simulink model "deep_fryer_adaptive_pid"  (R2024a)
settings: Solver=ode1  StartTime=0.0  StopTime=stop_time  FixedStep=dt  RelTol=1e-3
InitFcn:
  | if ~exist('tau','var'); tau = 180; end
  | if ~exist('L','var'); L = 10; end
  | if ~exist('K','var'); K = 1.9; end
  | if ~exist('T_ambient','var'); T_ambient = 30; end
  | if ~exist('Kp0','var'); Kp0 = 2; end
  | if ~exist('Ki0','var'); Ki0 = 0.05; end
  | if ~exist('Kd0','var'); Kd0 = 0.5; end
  | if ~exist('lambda_p','var'); lambda_p = 0.02; end
  | if ~exist('lambda_i','var'); lambda_i = 0.001; end
  | if ~exist('lambda_d','var'); lambda_d = 0.01; end
  | if ~exist('Kp_max','var'); Kp_max = 10; end
  | if ~exist('Ki_max','var'); Ki_max = 1; end
  | if ~exist('Kd_max','var'); Kd_max = 5; end
  | if ~exist('Tf_deriv','var'); Tf_deriv = 5; end
  | if ~exist('dead_hi','var'); dead_hi = 1.5; end
  | if ~exist('dead_lo','var'); dead_lo = 0.75; end
  | if ~exist('taper','var'); taper = 1; end
  | if ~exist('n_avg','var'); n_avg = 1; end
  | if ~exist('out_min','var'); out_min = 0; end
  | if ~exist('out_max','var'); out_max = 100; end
  | if ~exist('servo_tau','var'); servo_tau = 0.7; end
  | if ~exist('dt','var'); dt = 1; end
  | if ~exist('stop_time','var'); stop_time = 1800; end
  | if ~exist('Tref_value','var'); Tref_value = 150; end
values from neighbouring files (symbols this model uses):
  dead_hi = 1.5    [build_deep_fryer_model.m]
  dead_lo = 0.75    [build_deep_fryer_model.m]
  dt = 1    [build_deep_fryer_model.m]
  K = 1.9    [build_deep_fryer_model.m]
  Kd0 = 0.5    [build_deep_fryer_model.m]
  Kd_max = 5    [build_deep_fryer_model.m]
  Ki0 = 0.05    [build_deep_fryer_model.m]
  Ki_max = 1    [build_deep_fryer_model.m]
  Kp0 = 2    [build_deep_fryer_model.m]
  Kp_max = 10    [build_deep_fryer_model.m]
  L = 10    [build_deep_fryer_model.m]
  lambda_d = 0.01    [build_deep_fryer_model.m]
  lambda_i = 0.001    [build_deep_fryer_model.m]
  lambda_p = 0.02    [build_deep_fryer_model.m]
  n_avg = 1    [build_deep_fryer_model.m]
  out_max = 100    [build_deep_fryer_model.m]
  out_min = 0    [build_deep_fryer_model.m]
  servo_tau = 0.7    [build_deep_fryer_model.m]
  T_ambient = 30    [build_deep_fryer_model.m]
  taper = 1.0    (= 1)    [build_deep_fryer_model.m]
  tau = 180    [build_deep_fryer_model.m]
  Tf_deriv = 5    [build_deep_fryer_model.m]
  Tref_value = 150    [build_deep_fryer_model.m]
settings Model: Creator=indie  LastModifiedBy=indie

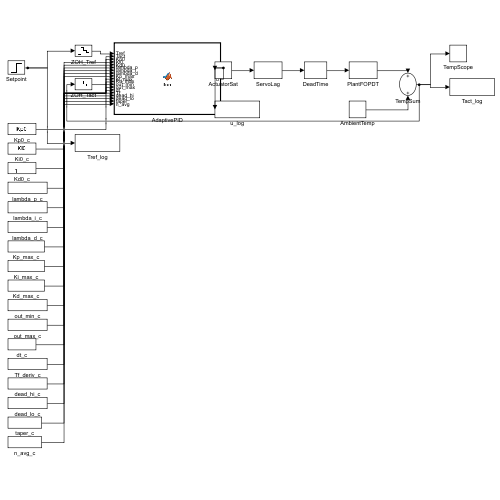
[thumbnail: Simulink's stored preview of the top-level diagram]
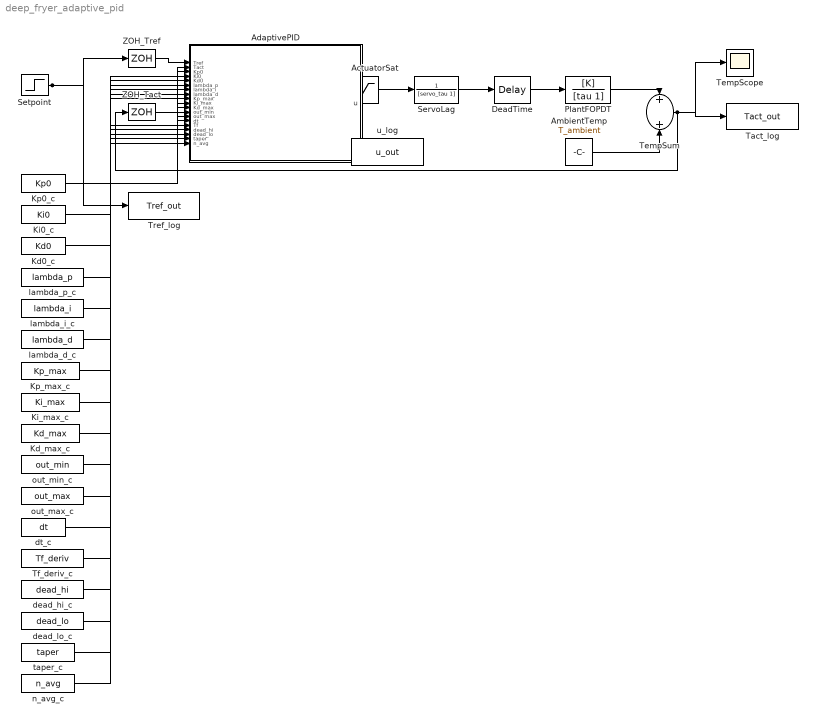
== system deep_fryer_adaptive_pid ==
  ActuatorSat : Saturate  UpperLimit=out_max  LowerLimit=out_min
  AdaptivePID : MATLAB Function  TreatAsAtomicUnit=on
  AmbientTemp : Constant  Value=T_ambient
  DeadTime : TransportDelay  DelayTime=L
  Kd0_c : Constant  Value=Kd0
  Kd_max_c : Constant  Value=Kd_max
  Ki0_c : Constant  Value=Ki0
  Ki_max_c : Constant  Value=Ki_max
  Kp0_c : Constant  Value=Kp0
  Kp_max_c : Constant  Value=Kp_max
  PlantFOPDT : TransferFcn  Numerator=[K]  Denominator=[tau 1]
  ServoLag : TransferFcn  Denominator=[servo_tau 1]
  Setpoint : Step  Time=0  Before=Tref_value  After=Tref_value  SampleTime=0
  Tact_log : ToWorkspace  VariableName=Tact_out  SaveFormat=Structure With Time  SampleTime=-1
  TempScope : Scope
  TempSum : Sum
  Tf_deriv_c : Constant  Value=Tf_deriv
  Tref_log : ToWorkspace  VariableName=Tref_out  SaveFormat=Structure With Time  SampleTime=-1
  ZOH_Tact : ZeroOrderHold  SampleTime=dt
  ZOH_Tref : ZeroOrderHold  SampleTime=dt
  dead_hi_c : Constant  Value=dead_hi
  dead_lo_c : Constant  Value=dead_lo
  dt_c : Constant  Value=dt
  lambda_d_c : Constant  Value=lambda_d
  lambda_i_c : Constant  Value=lambda_i
  lambda_p_c : Constant  Value=lambda_p
  n_avg_c : Constant  Value=n_avg
  out_max_c : Constant  Value=out_max
  out_min_c : Constant  Value=out_min
  taper_c : Constant  Value=taper
  u_log : ToWorkspace  VariableName=u_out  SaveFormat=Structure With Time  SampleTime=-1
  wires:
  ActuatorSat/1 -> ServoLag/1
  ServoLag/1 -> DeadTime/1
  DeadTime/1 -> PlantFOPDT/1
  PlantFOPDT/1 -> TempSum/1
  AmbientTemp/1 -> TempSum/2
  TempSum/1 -> TempScope/1, Tact_log/1, ZOH_Tact/1
  Setpoint/1 -> Tref_log/1, ZOH_Tref/1
  AdaptivePID/1(u) -> u_log/1, ActuatorSat/1
  ZOH_Tref/1 -> AdaptivePID/1(Tref)
  ZOH_Tact/1 -> AdaptivePID/2(Tact)
  Kp0_c/1 -> AdaptivePID/3(Kp0)
  Ki0_c/1 -> AdaptivePID/4(Ki0)
  Kd0_c/1 -> AdaptivePID/5(Kd0)
  lambda_p_c/1 -> AdaptivePID/6(lambda_p)
  lambda_i_c/1 -> AdaptivePID/7(lambda_i)
  lambda_d_c/1 -> AdaptivePID/8(lambda_d)
  Kp_max_c/1 -> AdaptivePID/9(Kp_max)
  Ki_max_c/1 -> AdaptivePID/10(Ki_max)
  Kd_max_c/1 -> AdaptivePID/11(Kd_max)
  out_min_c/1 -> AdaptivePID/12(out_min)
  out_max_c/1 -> AdaptivePID/13(out_max)
  dt_c/1 -> AdaptivePID/14(dt)
  Tf_deriv_c/1 -> AdaptivePID/15(Tf)
  dead_hi_c/1 -> AdaptivePID/16(dead_hi)
  dead_lo_c/1 -> AdaptivePID/17(dead_lo)
  taper_c/1 -> AdaptivePID/18(taper)
  n_avg_c/1 -> AdaptivePID/19(n_avg)

== matlab function deep_fryer_adaptive_pid/AdaptivePID ==
  data: Tref input; u output; Tact input; Kp0 input; Ki0 input; Kd0 input; lambda_p input; lambda_i input; lambda_d input; Kp_max input; Ki_max input; Kd_max input; out_min input; out_max input; dt input; Tf input; dead_hi input; dead_lo input; taper input; n_avg input
function u = adaptive_pid(Tref, Tact, Kp0, Ki0, Kd0, lambda_p, lambda_i, lambda_d, Kp_max, Ki_max, Kd_max, out_min, out_max, dt, Tf, dead_hi, dead_lo, taper, n_avg)
%#codegen
persistent e_prev sum_e d_filt initialized u_buf u_buf_idx buf_count
MAXN = 15;
if isempty(initialized)
    e_prev = 0;
    sum_e = 0;
    d_filt = 0;
    u_buf = zeros(1, MAXN);
    u_buf_idx = 0;
    buf_count = 0;
    initialized = true;
end

e = Tref - Tact;
delta_e = e - e_prev;

% -- derivative low-pass filter (first-order, time constant Tf) --
alpha = dt / (Tf + dt);
d_filt = d_filt + alpha * (delta_e/dt - d_filt);

Kp = min(Kp0 + lambda_p * abs(e), Kp_max);
Kd = min(Kd0 + lambda_d * abs(d_filt), Kd_max); % dijadwalkan dari d_filt (FIX #4), bukan delta_e mentah
Ki = min(Ki0 + lambda_i * abs(e), Ki_max); % dijadwalkan dari |e|, BUKAN |sum_e| -- lihat catatan FIX #2

% -- threshold asimetris: dead_hi (Tact di bawah Tref) vs dead_lo (Tact di atas Tref) --
inDeadband = (e <= dead_hi) && (e >= -dead_lo);

% -- gain tapering di dalam deadband (P & D tetap aktif, tidak dibekukan) --
if inDeadband
    Kp_eff = Kp * taper;
    Ki_eff = Ki * taper;
    Kd_eff = Kd * taper;
else
    Kp_eff = Kp;
    Ki_eff = Ki;
    Kd_eff = Kd;
end

% -- anti-windup: conditional integration (FIX #6) + deadband integral-only freeze --
sum_e_candidate = sum_e + e * dt;
u_candidate = Kp_eff*e + Ki_eff*sum_e_candidate + Kd_eff*d_filt;
if inDeadband
    doAccumulate = false; % Layer 1 -- TERBUKTI menghilangkan limit cycle, tidak diubah
elseif u_candidate > out_max
    doAccumulate = (e < 0); % izinkan integral MENGECIL (unwind) kalau error sudah berbalik
elseif u_candidate < out_min
    doAccumulate = (e > 0); % izinkan integral MEMBESAR kembali kalau error sudah berbalik
else
    doAccumulate = true;
end

if doAccumulate
    sum_e = sum_e_candidate;
    u_raw = u_candidate;
else
    u_raw = Kp_eff*e + Ki_eff*sum_e + Kd_eff*d_filt;
end
u_raw = min(max(u_raw, out_min), out_max);

% -- output averaging di dalam deadband (buffer sirkular ukuran MAXN) --
% FIX #7: hitung sample VALID (buf_count) supaya slot buffer yang
% belum pernah terisi (masih nol dari inisialisasi) tidak ikut
% dirata-rata dan menurunkan output secara tidak wajar.
u_buf_idx = mod(u_buf_idx, MAXN) + 1;
u_buf(u_buf_idx) = u_raw;
buf_count = min(buf_count + 1, MAXN);
if inDeadband && n_avg > 1
    nn = min([round(n_avg), MAXN, buf_count]);
    s = 0;
    for k = 0:(nn-1)
        pos = mod(u_buf_idx - 1 - k, MAXN) + 1;
        s = s + u_buf(pos);
    end
    u = s / nn;
else
    u = u_raw;
end

e_prev = e;
end
